simulink model "LoadTorque"  (R2025b)
settings: Solver=ode1  StartTime=0.0  StopTime=10.0  FixedStep=0.001  RelTol=1e-3
settings Model: Creator=williamvandevoir  LastModifiedBy=williamvandevoir

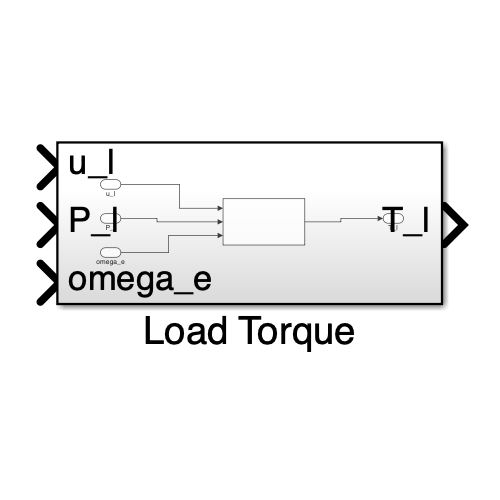
[thumbnail: Simulink's stored preview of the top-level diagram]
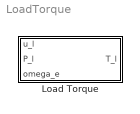
== system LoadTorque ==
  Load Torque : Subsystem

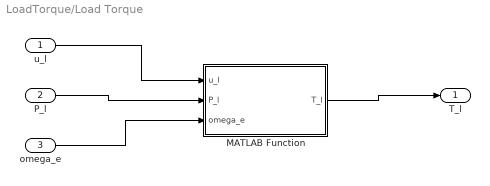
== system LoadTorque/Load Torque ==
  u_l : Inport
  P_l : Inport  Port=2
  omega_e : Inport  Port=3
  MATLAB Function : MATLAB Function  TreatAsAtomicUnit=on
  T_l : Outport
  wires:
  u_l/1 -> MATLAB Function/1(u_l)
  P_l/1 -> MATLAB Function/2(P_l)
  omega_e/1 -> MATLAB Function/3(omega_e)
  MATLAB Function/1(T_l) -> T_l/1

== matlab function LoadTorque/Load Torque/MATLAB Function ==
  data: u_l input; T_l output; P_l input; omega_e input; eta_gen parameter
function T_l = fcn(u_l, P_l, omega_e, eta_gen)
% Load torque: T_l = u_l * P_l / (omega_e * eta_gen)
% u_l: load on/off (1/0), P_l: load power [W], omega_e: engine speed [rad/s]
T_l = u_l * P_l / (omega_e * eta_gen);
